simulink model "Warning"  (R2024a)
settings: Solver=FixedStepDiscrete  StartTime=0.0  StopTime=WRN_Stop_Time  FixedStep=WRN_Step_Size  RelTol=1e-3  EnableMultiTasking=on
undefined symbols (not defined in the file): BSDState_T, LedState_T
settings Model: DataDictionary=bsd.sldd  Creator=pc  LastModifiedBy=pc
settings OptimizationCC: DefaultParameterBehavior=Inlined  UseDivisionForNetSlopeComputation=on  EnhancedBackFolding=on  PassReuseOutputArgsAs=Individual arguments  ZeroExternalMemoryAtStartup=off  ZeroInternalMemoryAtStartup=off  OptimizeBlockOrder=speed  DifferentSizesBufferReuse=on  OptimizationCustomize=off  EfficientTunableParamExpr=on
settings DebuggingCC: ParameterTunabilityLossMsg=error
settings SFSimCC: MATLABDynamicMemAlloc=off
settings RTWCC: Description=AUTOSAR  SystemTargetFile=autosar.tlc  GenCodeOnly=on  TemplateMakefile=ert_default_tmf  DataTypeReplacement=CDataTypesFixedWidth
settings CodeAppCC: ForceParamTrailComments=on  IgnoreCustomStorageClasses=off  OperatorAnnotations=on  SimulinkDataObjDesc=on  SFDataObjDesc=on  InsertBlockDesc=on
settings STFCustomTargetCC: MultiwordLength=256  ParMdlRefBuildCompliant=on  CompOptLevelCompliant=on  IncludeMdlTerminateFcn=off  CombineOutputUpdateFcns=on  SuppressErrorStatus=on  ERTCustomFileBanners=on  SupportNonFinite=off  SupportComplex=off  SupportContinuousTime=off  SupportNonInlinedSFcns=off  RemoveResetFunc=on  MATLABClassNameForMDSCustomization=Simulink.SoftwareTarget.ERTCustomization  AutosarCompliant=on  GRTInterface=off  LookupTableObjectStructAxisOrder=2,1,3,4,...  LUTObjectStructOrderEvenSpacing=Size,Table,Breakpoints  SystemTargetFile=autosar.tlc
settings ERTTargetCC: TargetLangStandard=C99 (ISO)  ConcurrentExecutionCompliant=off  IncludeMdlTerminateFcn=off  SuppressErrorStatus=on  SupportNonFinite=off  SupportComplex=off  ModelStepFunctionPrototypeControlCompliant=off  CPPClassGenCompliant=off  AutosarCompliant=on  LookupTableObjectStructAxisOrder=2,1,3,4,...  LUTObjectStructOrderEvenSpacing=Size,Table,Breakpoints  InlinedParameterPlacement=NonHierarchical  ERTCustomFileTemplate=example_file_process.tlc  BooleanTrueId=TRUE  BooleanFalseId=FALSE

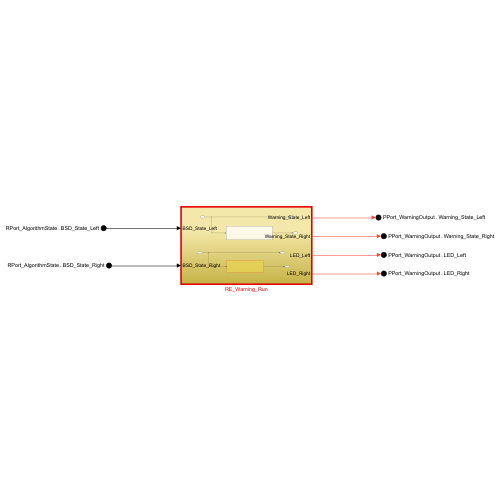
[thumbnail: Simulink's stored preview of the top-level diagram]
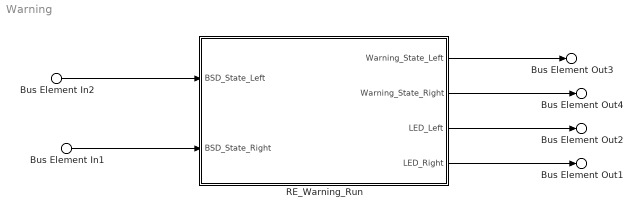
== system Warning ==
  Bus Element In1 : Inport  PortName=RPort_AlgorithmState  Element=BSD_State_Right
  Bus Element In2 : Inport  PortName=RPort_AlgorithmState  Element=BSD_State_Left
  RE_Warning_Run : Subsystem  TreatAsAtomicUnit=on
  Bus Element Out1 : Outport  PortName=PPort_WarningOutput  Element=LED_Right
  Bus Element Out2 : Outport  PortName=PPort_WarningOutput  Element=LED_Left
  Bus Element Out3 : Outport  PortName=PPort_WarningOutput  Element=Warning_State_Left
  Bus Element Out4 : Outport  PortName=PPort_WarningOutput  Element=Warning_State_Right
  wires:
  Bus Element In1/1 -> RE_Warning_Run/2(BSD_State_Right)
  Bus Element In2/1 -> RE_Warning_Run/1(BSD_State_Left)
  RE_Warning_Run/4(LED_Right) -> Bus Element Out1/1
  RE_Warning_Run/3(LED_Left) -> Bus Element Out2/1
  RE_Warning_Run/1(Warning_State_Left) -> Bus Element Out3/1
  RE_Warning_Run/2(Warning_State_Right) -> Bus Element Out4/1

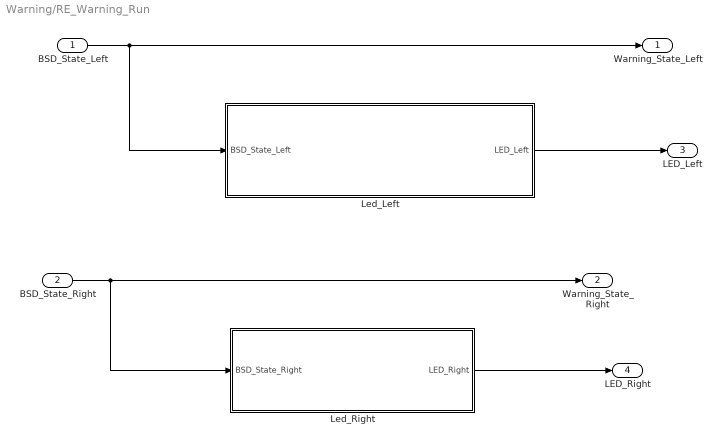
== system Warning/RE_Warning_Run ==
  BSD_State_Left : Inport  OutDataTypeStr=Enum: BSDState_T
  BSD_State_Right : Inport  Port=2  OutDataTypeStr=Enum: BSDState_T
  Led_Left : Subsystem
  Led_Right : Subsystem
  Warning_State_Left : Outport  OutDataTypeStr=Enum: BSDState_T
  Warning_State_Right : Outport  Port=2  OutDataTypeStr=Enum: BSDState_T
  LED_Left : Outport  Port=3  OutDataTypeStr=Enum: LedState_T
  LED_Right : Outport  Port=4  OutDataTypeStr=Enum: LedState_T
  wires:
  BSD_State_Left/1 -> Led_Left/1(BSD_State_Left), Warning_State_Left/1
  BSD_State_Right/1 -> Led_Right/1(BSD_State_Right), Warning_State_Right/1
  Led_Left/1(LED_Left) -> LED_Left/1
  Led_Right/1(LED_Right) -> LED_Right/1

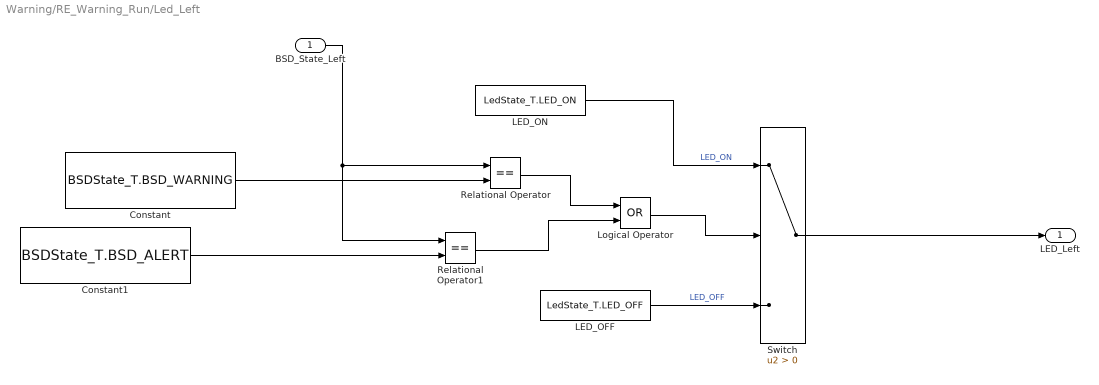
== system Warning/RE_Warning_Run/Led_Left ==
  BSD_State_Left : Inport
  Constant : Constant  Value=BSDState_T.BSD_WARNING  OutDataTypeStr=Enum: BSDState_T
  Constant1 : Constant  Value=BSDState_T.BSD_ALERT  OutDataTypeStr=Enum: BSDState_T
  LED_OFF : Constant  Value=LedState_T.LED_OFF  OutDataTypeStr=Enum: LedState_T
  LED_ON : Constant  Value=LedState_T.LED_ON  OutDataTypeStr=Enum: LedState_T
  Logical Operator : Logic  Operator=OR  AllPortsSameDT=off  OutDataTypeStr=boolean
  Relational Operator : RelationalOperator  Operator===  OutDataTypeStr=boolean  RndMeth=Simplest  InputSameDT=off
  Relational Operator1 : RelationalOperator  Operator===  OutDataTypeStr=boolean  RndMeth=Simplest  InputSameDT=off
  Switch : Switch  Criteria=u2 > Threshold  SaturateOnIntegerOverflow=off  InputSameDT=off
  LED_Left : Outport  OutDataTypeStr=Enum: LedState_T
  wires:
  Constant/1 -> Relational Operator/2
  Constant1/1 -> Relational Operator1/2
  Logical Operator/1 -> Switch/2
  BSD_State_Left/1 -> Relational Operator1/1, Relational Operator/1
  Relational Operator1/1 -> Logical Operator/2
  Relational Operator/1 -> Logical Operator/1
  LED_OFF/1 -> Switch/3  "LED_OFF"
  LED_ON/1 -> Switch/1  "LED_ON"
  Switch/1 -> LED_Left/1

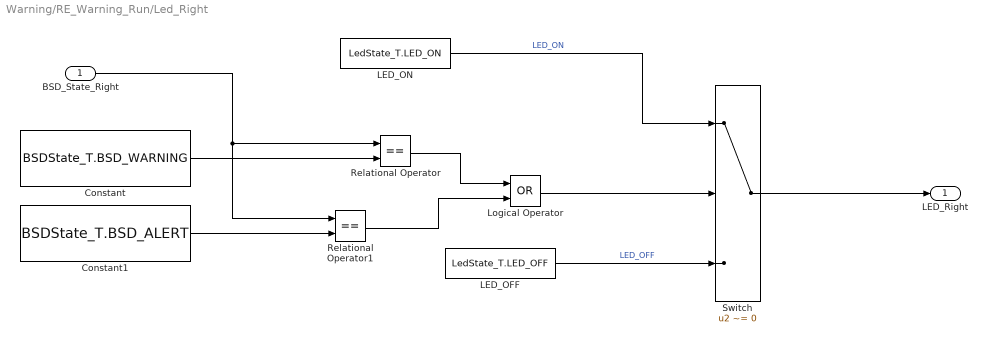
== system Warning/RE_Warning_Run/Led_Right ==
  BSD_State_Right : Inport
  Constant : Constant  Value=BSDState_T.BSD_WARNING  OutDataTypeStr=Enum: BSDState_T
  Constant1 : Constant  Value=BSDState_T.BSD_ALERT  OutDataTypeStr=Enum: BSDState_T
  LED_OFF : Constant  Value=LedState_T.LED_OFF  OutDataTypeStr=Enum: LedState_T
  LED_ON : Constant  Value=LedState_T.LED_ON  OutDataTypeStr=Enum: LedState_T
  Logical Operator : Logic  Operator=OR  AllPortsSameDT=off  OutDataTypeStr=boolean
  Relational Operator : RelationalOperator  Operator===  OutDataTypeStr=boolean  RndMeth=Simplest  InputSameDT=off
  Relational Operator1 : RelationalOperator  Operator===  OutDataTypeStr=boolean  RndMeth=Simplest  InputSameDT=off
  Switch : Switch  Criteria=u2 ~= 0  SaturateOnIntegerOverflow=off  InputSameDT=off
  LED_Right : Outport  OutDataTypeStr=Enum: LedState_T
  wires:
  Relational Operator/1 -> Logical Operator/1
  Relational Operator1/1 -> Logical Operator/2
  Switch/1 -> LED_Right/1
  BSD_State_Right/1 -> Relational Operator/1, Relational Operator1/1
  Logical Operator/1 -> Switch/2
  Constant1/1 -> Relational Operator1/2
  Constant/1 -> Relational Operator/2
  LED_ON/1 -> Switch/1  "LED_ON"
  LED_OFF/1 -> Switch/3  "LED_OFF"
